simulink model "SafetyMonitor"  (R2025b)
settings: Solver=VariableStepAuto  StartTime=0.0  StopTime=10.0  RelTol=1e-3
settings Model: Creator=Ishwar  LastModifiedBy=Ishwar

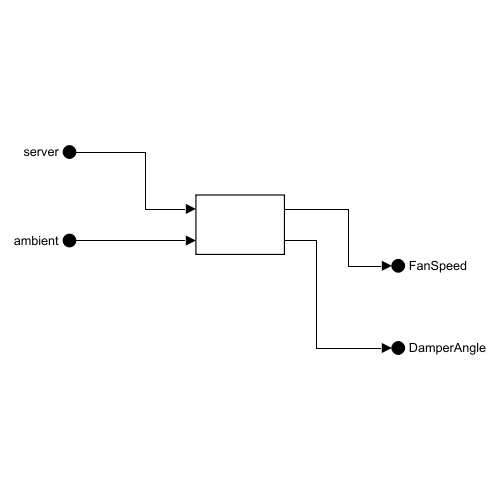
[thumbnail: Simulink's stored preview of the top-level diagram]
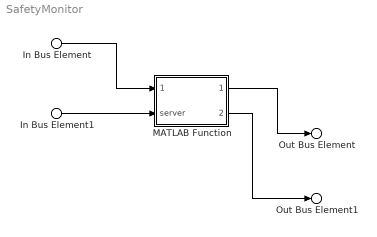
== system SafetyMonitor ==
  In Bus Element : Inport  PortName=server
  In Bus Element1 : Inport  Port=2  PortName=ambient
  MATLAB Function : MATLAB Function  TreatAsAtomicUnit=on
  Out Bus Element : Outport  PortName=FanSpeed
  Out Bus Element1 : Outport  Port=2  PortName=DamperAngle
  wires:
  In Bus Element1/1 -> MATLAB Function/2(server)
  In Bus Element/1 -> MATLAB Function/1(ambient)
  MATLAB Function/1(FanSpeed) -> Out Bus Element/1
  MATLAB Function/2(DamperAngle) -> Out Bus Element1/1

== matlab function SafetyMonitor/MATLAB Function ==
  data: ambient input; FanSpeed output; server input; DamperAngle output
function [FanSpeed, DamperAngle] = SafetyMonitor(ambient, server)
%#codegen
maxServerTemp = 75;   % °C
maxAmbientTemp = 45;  % °C

% Default safe values
FanSpeed = 50;        % moderate cooling
DamperAngle = 30;     % partially open

% Escalate if temperatures exceed thresholds
if server > maxServerTemp || ambient > maxAmbientTemp
    FanSpeed = 100;       % full cooling
    DamperAngle = 90;     % fully open
end
